simulink model "FullFMS_SIM_V0_1_0_R2025b"  (R2025b)
settings: Solver=FixedStepAuto  StopTime=inf  FixedStep=0.01  MaxStep=0.01  RelTol=1e-2
PreLoadFcn:
  | load("BUS_CONFIG_SIM.mat"); run("Param_SIM_V0_6.m")
values from neighbouring files (symbols this model uses):
  N_PARTS = 3    [Param_SIM_V0_1_2.m]    (also in Param_SIM_V0_1_3.m; Param_SIM_V0_1_4.m; Param_SIM_V0_1_5.m; Param_SIM_V0_1_6.m)
  t_conv = 5    [Param_SIM_V0_1_2.m]    (also in Param_SIM_V0_1_3.m; Param_SIM_V0_1_4.m; Param_SIM_V0_1_5.m; Param_SIM_V0_1_6.m)
  T_CONV_T6 = 3    [Param_SIM_V0_1_2.m]    (also in Param_SIM_V0_1_3.m; Param_SIM_V0_1_4.m; Param_SIM_V0_1_5.m; Param_SIM_V0_1_6.m)
  t_grip = 0.10    (= 0.1)    [Param_SIM_V0_1_2.m]    (also in Param_SIM_V0_1_3.m; Param_SIM_V0_1_4.m; Param_SIM_V0_1_5.m; Param_SIM_V0_1_6.m)
  t_h_cart = 2.38    [Param_SIM_V0_1_2.m]    (also in Param_SIM_V0_1_3.m; Param_SIM_V0_1_4.m; Param_SIM_V0_1_5.m; Param_SIM_V0_1_6.m)
  t_h_del = 2.82    [Param_SIM_V0_1_2.m]    (also in Param_SIM_V0_1_3.m; Param_SIM_V0_1_4.m; Param_SIM_V0_1_5.m; Param_SIM_V0_1_6.m)
  T_HD1_T1 = 2    [Param_SIM_V0_1_2.m]    (also in Param_SIM_V0_1_3.m; Param_SIM_V0_1_4.m; Param_SIM_V0_1_5.m; Param_SIM_V0_1_6.m)
  t_leave = 2    [Param_SIM_V0_1_2.m]    (also in Param_SIM_V0_1_3.m; Param_SIM_V0_1_4.m; Param_SIM_V0_1_5.m; Param_SIM_V0_1_6.m)
  t_sort_clear = 3    [Param_SIM_V0_6.m]
  t_v_down = 0.93    [Param_SIM_V0_1_2.m]    (also in Param_SIM_V0_1_3.m; Param_SIM_V0_1_4.m; Param_SIM_V0_1_5.m; Param_SIM_V0_1_6.m)
  t_v_up = 1.37    [Param_SIM_V0_1_2.m]    (also in Param_SIM_V0_1_3.m; Param_SIM_V0_1_4.m; Param_SIM_V0_1_5.m; Param_SIM_V0_1_6.m)
libraries: opcualib x8
settings Model: SimulationMode=accelerator  PacingRate=0.100000  Creator=guilh  LastModifiedBy=gasie
settings SolverCC: ZeroCrossControl=DisableAll

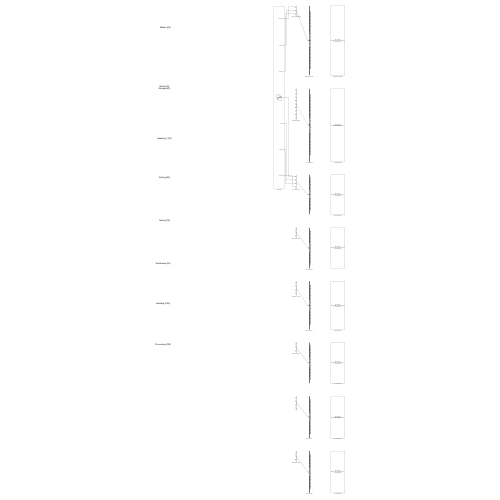
[thumbnail: Simulink's stored preview of the top-level diagram]
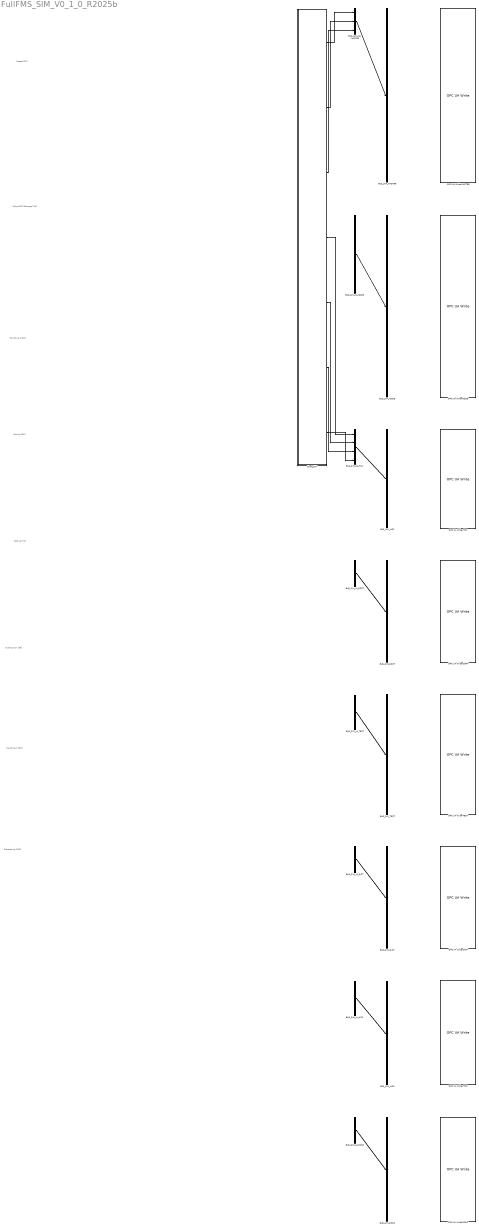
== system FullFMS_SIM_V0_1_0_R2025b ==
  note: Master [20]
  note: Robot [30]
      | Storage [40]
  note: Handling 1 [50]
  note: Sorting [60]
  note: Testing [70]
  note: Distribution [80]
  note: Handling 2 [90]
  note: Processing [100]
  BUS_SIM_DIST : BusSelector  OutputSignals=SimActuators_80.SA_80_Pist_Adv,SimActuators_80.SA_80_Suction_On,SimActuators_80.SA_80_Suction_Off,SimActuators_80.SA_80_Arm_2_Del,SimActuators_80.SA_80_Arm_2_Mag,SimActuators_80.SA_81_Led_Start,SimActuators_80.SA_81_Led_Reset,SimActuators_80.SA_81_Led_Extra1,SimActuators_80.SA_81_Led_Extra2,SimActuators_80.SA_81_Panel_O4,SimActuators_80.SA_81_Panel_O5,SimActuators_80.SA_81_Panel_O6,SimActuators_80.SA_81_Panel_O7,SimControl_80.SC_82_Profibus,SimControl_80.SC_83_RQ_Parts,SimControl_80.SC_85_Initialization,SimControl_80.SC_85_Start,SimControl_80.SC_85_Part_Del,SimControl_80.SC_85_Single,SimControl_80.SC_85_Part_Mag,SimControl_80.SC_85_Continuous,SimControl_80.SC_85_Counted,SimControl_80.SC_86_Mag_Parts,SimControl_80.SC_87_RQ_MParts,SimSensors_80.SS_80_Mag_Full,SimSensors_80.SS_80_Pist_Bck,SimSensors_80.SS_80_Pist_Fwd,SimSensors_80.SS_80_Part_Stuck,SimSensors_80.SS_80_Arm_Mag,SimSensors_80.SS_80_Arm_Del,SimSensors_80.SS_80_Mag_Empty,SimSensors_80.SS_81_Start,SimSensors_80.SS_81_Stop,SimSensors_80.SS_81_Key_Pos,SimSensors_80.SS_81_Reset,SimSensors_80.SS_81_Panel_I4,SimSensors_80.SS_81_Panel_I5,SimSensors_80.SS_81_Panel_I6,SimSensors_80.SS_81_Panel_I7
  BUS_SIM_HD1 : BusSelector  OutputSignals=SimActuators_50.SA_50_Claw_2_Del,SimActuators_50.SA_50_Claw_2_Cart,SimActuators_50.SA_50_Claw_Down,SimActuators_50.SA_50_Close_Claw,SimActuators_50.SA_51_Led_Start,SimActuators_50.SA_51_Led_Reset,SimActuators_50.SA_51_Led_Extra1,SimActuators_50.SA_51_Led_Extra2,SimActuators_50.SA_51_Panel_O4,SimActuators_50.SA_51_Panel_O5,SimActuators_50.SA_51_Panel_O6,SimActuators_50.SA_51_Panel_O7,SimASi_50.SR_53_SortCartID,SimASi_50.SR_54_Request,SimASi_50.SR_54_No_Cart,SimASi_50.SR_54_Cart_Full,SimASi_50.SR_54_CRoute_Out,SimASi_50.SR_54_CRoute_In,SimControl_50.SC_52_Profibus,SimControl_50.SC_55_Initialization,SimControl_50.SC_55_Start,SimControl_50.SC_55_PD_Sort,SimControl_50.SC_55_Cart2Del,SimSensors_50.SS_50_Part_Reserve,SimSensors_50.SS_50_Claw_Cart,SimSensors_50.SS_50_Claw_Del,SimSensors_50.SS_50_Claw_Reserve,SimSensors_50.SS_50_Claw_Low,SimSensors_50.SS_50_Claw_High,SimSensors_50.SS_50_Part_in_Claw,SimSensors_50.SS_51_Start,SimSensors_50.SS_51_Stop,SimSensors_50.SS_51_Key_Pos,SimSensors_50.SS_51_Reset,SimSensors_50.SS_51_Panel_I4,SimSensors_50.SS_51_Panel_I5,SimSensors_50.SS_51_Panel_I6,SimSensors_50.SS_51_Panel_I7
  BUS_SIM_HD2 : BusSelector  OutputSignals=SimActuators_90.SA_90_Claw_2_Cart,SimActuators_90.SA_90_Claw_2_Del,SimActuators_90.SA_90_Claw_Down,SimActuators_90.SA_90_Close_Claw,SimActuators_90.SA_91_Led_Start,SimActuators_90.SA_91_Led_Reset,SimActuators_90.SA_91_Led_Extra1,SimActuators_90.SA_91_Led_Extra2,SimActuators_90.SA_91_Panel_O4,SimActuators_90.SA_91_Panel_O5,SimActuators_90.SA_91_Panel_O6,SimActuators_90.SA_91_Panel_O7,SimASi_90.SR_93_ProcCartID,SimASi_90.SR_94_Request,SimASi_90.SR_94_No_Cart,SimASi_90.SR_94_Cart_Full,SimASi_90.SR_94_CRoute_Out,SimASi_90.SR_94_CRoute_In,SimControl_90.SC_92_Profibus,SimControl_90.SC_95_Initialization,SimControl_90.SC_95_Start,SimControl_90.SC_95_PD_Proc,SimControl_90.SC_95_Cart2Del,SimControl_90.SC_95_PD_Cart,SimControl_90.SC_95_Del2Cart,SimSensors_90.SS_90_Part_Reserve,SimSensors_90.SS_90_Claw_Del,SimSensors_90.SS_90_Claw_Cart,SimSensors_90.SS_90_Claw_Reserve,SimSensors_90.SS_90_Claw_Low,SimSensors_90.SS_90_Claw_High,SimSensors_90.SS_90_Part_in_Claw,SimSensors_90.SS_91_Start,SimSensors_90.SS_91_Stop,SimSensors_90.SS_91_Key_Pos,SimSensors_90.SS_91_Reset,SimSensors_90.SS_91_Panel_I4,SimSensors_90.SS_91_Panel_I5,SimSensors_90.SS_91_Panel_I6,SimSensors_90.SS_91_Panel_I7
  BUS_SIM_IN_DIST : BusCreator  Inputs=3  OutDataTypeStr=Bus: B_SIM_DIST  NonVirtualBus=on
  BUS_SIM_IN_HD1 : BusCreator  Inputs=4  OutDataTypeStr=Bus: B_SIM_HD1  NonVirtualBus=on
  BUS_SIM_IN_HD2 : BusCreator  Inputs=4  OutDataTypeStr=Bus: B_SIM_HD2  NonVirtualBus=on
  BUS_SIM_IN_MASTER : BusCreator  Inputs=3  OutDataTypeStr=Bus: B_SIM_MASTER  NonVirtualBus=on
  BUS_SIM_IN_NODE : BusCreator  Inputs=9  OutDataTypeStr=Bus: B_SIM_NODE  NonVirtualBus=on
  BUS_SIM_IN_PROC : BusCreator  Inputs=3  OutDataTypeStr=Bus: B_SIM_PROC  NonVirtualBus=on
  BUS_SIM_IN_SORT : BusCreator  Inputs=3  OutDataTypeStr=Bus: B_SIM_SORT  NonVirtualBus=on
  BUS_SIM_IN_TEST : BusCreator  Inputs=4  OutDataTypeStr=Bus: B_SIM_TEST  NonVirtualBus=on
  BUS_SIM_MASTER : BusSelector  OutputSignals=SimActuators_20.SA_20_Led_On,SimActuators_20.SA_20_Led_Off,SimActuators_20.SA_20_Conveyor,SimActuators_20.SA_24_Cart_Test,SimActuators_20.SA_25_Cart_Proc,SimActuators_20.SA_26_Cart_Visi,SimActuators_20.SA_27_Cart_Robo,SimActuators_20.SA_28_Cart_Stor,SimActuators_20.SA_29_Cart_Sort,SimControl_20.SC_21_MES_On,SimControl_20.SC_24_Request,SimControl_20.SC_24_CRoute_In,SimControl_20.SC_24_CartDel,SimControl_20.SC_24_CRoute_Out,SimControl_20.SC_25_Request,SimControl_20.SC_25_CRoute_In,SimControl_20.SC_25_CartDel,SimControl_20.SC_25_CRoute_Out,SimControl_20.SC_26_Request,SimControl_20.SC_26_CRoute_In,SimControl_20.SC_26_CartDel,SimControl_20.SC_26_CRoute_Out,SimControl_20.SC_27_Request,SimControl_20.SC_27_CRoute_In,SimControl_20.SC_27_CartDel,SimControl_20.SC_27_CRoute_Out,SimControl_20.SC_28_Request,SimControl_20.SC_28_CRoute_In,SimControl_20.SC_28_CartDel,SimControl_20.SC_28_CRoute_Out,SimControl_20.SC_29_Request,SimControl_20.SC_29_CRoute_In,SimControl_20.SC_29_CartDel,SimControl_20.SC_29_CRoute_Out,SimSensors_20.SS_20_On,SimSensors_20.SS_20_Off,SimSensors_20.SS_20_Controler_On,SimSensors_20.SS_24_Cart_Stat,SimSensors_20.SS_24_Cart_Next,SimSensors_20.SS_24_Optic,SimSensors_20.SS_24_Count,SimSensors_20.SS_24_Pist_Bck,SimSensors_20.SS_25_Cart_Stat,SimSensors_20.SS_25_Cart_Next,SimSensors_20.SS_25_Optic,SimSensors_20.SS_25_Count,SimSensors_20.SS_25_Pist_Bck,SimSensors_20.SS_26_Cart_Stat,SimSensors_20.SS_26_Cart_Next,SimSensors_20.SS_26_Optic,SimSensors_20.SS_26_Count,SimSensors_20.SS_26_Pist_Bck,SimSensors_20.SS_27_Cart_Stat,SimSensors_20.SS_27_Cart_Next,SimSensors_20.SS_27_Optic,SimSensors_20.SS_27_Count,SimSensors_20.SS_27_Pist_Bck,SimSensors_20.SS_28_Cart_Stat,SimSensors_20.SS_28_Cart_Next,SimSensors_20.SS_28_Optic,SimSensors_20.SS_28_Count,SimSensors_20.SS_28_Pist_Bck,SimSensors_20.SS_29_Cart_Stat,SimSensors_20.SS_29_Cart_Next,SimSensors_20.SS_29_Optic,SimSensors_20.SS_29_Count,SimSensors_20.SS_29_Pist_Bck
  BUS_SIM_NODE : BusSelector  OutputSignals=SimActuators_30.SA_30_Led_Start,SimActuators_30.SA_30_Led_Reset,SimActuators_30.SA_30_Led_Extra1,SimActuators_30.SA_30_Led_Extra2,SimActuators_30.SA_30_Spring_Cyl,SimActuators_30.SA_30_Cover_Cyl,SimASi_30.SR_32_RoboCartID,SimASi_30.SR_34_Request,SimASi_30.SR_34_No_Cart,SimASi_30.SR_34_Cart_Full,SimASi_30.SR_34_CRoute_Out,SimASi_30.SR_34_CRoute_In,SimControl_30.SC_30_Robot1,SimControl_30.SC_30_Robot2,SimControl_30.SC_35_Part_Del,SimSensors_30.SS_31_Start,SimSensors_30.SS_31_Stop,SimSensors_30.SS_31_Reset,SimSensors_30.SS_31_Part_in_Claw,SimSensors_30.SS_31_Orientation,SimSensors_30.SS_32_Sp_Cyl_Bck,SimSensors_30.SS_32_Sp_Cyl_Fwd,SimSensors_30.SS_32_Co_Cyl_Bck,SimSensors_30.SS_32_Co_Cyl_Fwd,SimSensors_30.SS_32_Sp_PickUp,SimSensors_30.SS_32_Co_PickUp,SimSensors_30.SS_32_CoMag_Empty,SimRFID_RFID.SID_Ant1_R_TagID,SimRFID_RFID.SID_Ant1_R_UserData,SimRFID_RFID.SID_Ant1_W_TagID,SimRFID_RFID.SID_Ant1_W_UserData,SimRFID_RFID.SID_Ant2_R_TagID,SimRFID_RFID.SID_Ant2_R_UserData,SimRFID_RFID.SID_Ant2_W_TagID,SimRFID_RFID.SID_Ant2_W_UserData,SimRFID_RFID.SID_Ant3_R_TagID,SimRFID_RFID.SID_Ant3_R_UserData,SimRFID_RFID.SID_Ant3_W_TagID,SimRFID_RFID.SID_Ant3_W_UserData,SimRFID_RFID.SID_Ant4_R_TagID,SimRFID_RFID.SID_Ant4_R_UserData,SimRFID_RFID.SID_Ant4_W_TagID,SimRFID_RFID.SID_Ant4_W_UserData,SimActuators_40.SA_41_Led_Start,SimActuators_40.SA_41_Led_Reset,SimActuators_40.SA_41_Led_Extra1,SimActuators_40.SA_41_Led_Extra2,SimActuators_40.SA_41_Panel_O4,SimActuators_40.SA_41_Panel_O5,SimActuators_40.SA_41_Panel_O6,SimActuators_40.SA_41_Panel_O7,SimASi_40.SR_43_StorCartID,SimASi_40.SR_44_Request,SimASi_40.SR_44_No_Cart,SimASi_40.SR_44_Cart_Full,SimASi_40.SR_44_CRoute_Out,SimASi_40.SR_44_CRoute_In,SimControl_40.SC_42_Profibus,SimControl_40.SC_45_Initialization,SimControl_40.SC_45_Start,SimControl_40.SC_45_StorePart,SimControl_40.SC_45_RetrievePart,SimSensors_40.SS_41_Start,SimSensors_40.SS_41_Stop,SimSensors_40.SS_41_Key_Pos,SimSensors_40.SS_41_Reset,SimSensors_40.SS_41_Panel_I4,SimSensors_40.SS_41_Panel_I5,SimSensors_40.SS_41_Panel_I6,SimSensors_40.SS_41_Panel_I7
  BUS_SIM_PROC : BusSelector  OutputSignals=SimActuators_100.SA_100_Drill_On,SimActuators_100.SA_100_RT_On,SimActuators_100.SA_100_Drill_Down,SimActuators_100.SA_100_Drill_Up,SimActuators_100.SA_100_Drill_Pin,SimActuators_100.SA_100_Test_Pin,SimActuators_100.SA_101_Led_Start,SimActuators_100.SA_101_Led_Reset,SimActuators_100.SA_101_Led_Extra1,SimActuators_100.SA_101_Led_Extra2,SimActuators_100.SA_101_Panel_O4,SimActuators_100.SA_101_Panel_O5,SimActuators_100.SA_101_Panel_O6,SimActuators_100.SA_101_Panel_O7,SimControl_100.SC_102_Profibus,SimControl_100.SC_103_RQ_Turns,SimControl_100.SC_105_Initialization,SimControl_100.SC_105_Start,SimControl_100.SC_105_Part_ready,SimControl_100.SC_105_Test,SimControl_100.SC_105_Test_Ok,SimControl_100.SC_105_TestDrill,SimControl_100.SC_105_Test_Fail,SimControl_100.SC_105_Rotation,SimControl_100.SC_106_RT_Counter,SimSensors_100.SS_100_PInit_Pos,SimSensors_100.SS_100_PDrill_Pos,SimSensors_100.SS_100_PTest_Pos,SimSensors_100.SS_100_SDrill_High,SimSensors_100.SS_100_SDrill_Low,SimSensors_100.SS_100_RT_Sensor,SimSensors_100.SS_100_PTest_Ok,SimSensors_100.SS_101_Start,SimSensors_100.SS_101_Stop,SimSensors_100.SS_101_Key_Pos,SimSensors_100.SS_101_Reset,SimSensors_100.SS_101_Panel_I4,SimSensors_100.SS_101_Panel_I5,SimSensors_100.SS_101_Panel_I6,SimSensors_100.SS_101_Panel_I7
  BUS_SIM_SORT : BusSelector  OutputSignals=SimActuators_60.SA_60_Conveyor,SimActuators_60.SA_60_P1,SimActuators_60.SA_60_P2,SimActuators_60.SA_60_Identify,SimActuators_60.SA_61_Led_Start,SimActuators_60.SA_61_Led_Reset,SimActuators_60.SA_61_Led_Extra1,SimActuators_60.SA_61_Led_Extra2,SimActuators_60.SA_61_Panel_O4,SimActuators_60.SA_61_Panel_O5,SimActuators_60.SA_61_Panel_O6,SimActuators_60.SA_61_Panel_O7,SimControl_60.SC_62_Profibus,SimControl_60.SC_65_Initialization,SimControl_60.SC_65_RBS_Output,SimControl_60.SC_65_ID_1,SimControl_60.SC_65_RSB_Output,SimControl_60.SC_65_ID_2,SimControl_60.SC_65_BRS_Output,SimControl_60.SC_65_Part_Sorted,SimControl_60.SC_65_BSR_Output,SimControl_60.SC_65_SRB_Output,SimControl_60.SC_65_SBR_Output,SimSensors_60.SS_60_SPart,SimSensors_60.SS_60_SInd,SimSensors_60.SS_60_SPhoto,SimSensors_60.SS_60_Part_Pass,SimSensors_60.SS_60_SL1_Bck,SimSensors_60.SS_60_SL1_Fwd,SimSensors_60.SS_60_SL2_Bck,SimSensors_60.SS_60_SL2_Fwd,SimSensors_60.SS_61_Start,SimSensors_60.SS_61_Stop,SimSensors_60.SS_61_Key_Pos,SimSensors_60.SS_61_Reset,SimSensors_60.SS_61_Panel_I4,SimSensors_60.SS_61_Panel_I5,SimSensors_60.SS_61_Panel_I6,SimSensors_60.SS_61_Panel_I7
  BUS_SIM_TEST : BusSelector  OutputSignals=SimActuators_70.SA_70_Elev_Down,SimActuators_70.SA_70_Elev_Up,SimActuators_70.SA_70_Eject_Part,SimActuators_70.SA_70_Air_On,SimActuators_70.SA_71_Led_Start,SimActuators_70.SA_71_Led_Reset,SimActuators_70.SA_71_Led_Extra1,SimActuators_70.SA_71_Led_Extra2,SimActuators_70.SA_71_Panel_O4,SimActuators_70.SA_71_Panel_O5,SimActuators_70.SA_71_Panel_O6,SimActuators_70.SA_71_Panel_O7,SimASi_70.SR_73_TestCartID,SimASi_70.SR_74_Request,SimASi_70.SR_74_No_Cart,SimASi_70.SR_74_Cart_Full,SimASi_70.SR_74_CRoute_Out,SimASi_70.SR_74_CRoute_In,SimControl_70.SC_72_Profibus,SimControl_70.SC_75_Initialization,SimControl_70.SC_75_RQ_Delivery1,SimControl_70.SC_75_ID_Delivery1,SimControl_70.SC_75_RQ_Delivery2,SimControl_70.SC_75_ID_Delivery2,SimControl_70.SC_75_Identified,SimControl_70.SC_75_Part_Del,SimControl_70.SC_75_Requested,SimControl_70.SC_75_RQ_Part_Del,SimControl_70.SC_75_RQ_Wrong,SimControl_70.SC_75_Identified80,SimControl_70.SC_75_Requested80,SimSensors_70.SS_70_SInductive,SimSensors_70.SS_70_SPart,SimSensors_70.SS_70_SStation,SimSensors_70.SS_70_SPart_Height,SimSensors_70.SS_70_Elev_High,SimSensors_70.SS_70_Elev_Low,SimSensors_70.SS_70_Pist_Bck,SimSensors_70.SS_71_Start,SimSensors_70.SS_71_Stop,SimSensors_70.SS_71_Key_Pos,SimSensors_70.SS_71_Reset,SimSensors_70.SS_71_Panel_I4,SimSensors_70.SS_71_Panel_I5,SimSensors_70.SS_71_Panel_I6,SimSensors_70.SS_71_Panel_I7
  Chart_SIM : Stateflow chart  TreatAsAtomicUnit=on
  OPC UA Write-DIST : opcualib/OPC UA Write  SelectedServer=AAS OPC Distribution  ServerList=AAS OPC Distribution  NodeList={}  SampleTime=-1
  OPC UA Write-HD1 : opcualib/OPC UA Write  SelectedServer=AAS OPC Handling1  ServerList=AAS OPC Handling1  NodeList={}  SampleTime=-1
  OPC UA Write-HD2 : opcualib/OPC UA Write  SelectedServer=AAS OPC Handling2  ServerList=AAS OPC Handling2  NodeList={}  SampleTime=-1
  OPC UA Write-MASTER : opcualib/OPC UA Write  SelectedServer=AAS OPC Master  ServerList=AAS OPC Master  NodeList={}  SampleTime=-1
  OPC UA Write-NODE : opcualib/OPC UA Write  SelectedServer=AAS Server Robot+Storage  ServerList=AAS Server Robot+Storage  NodeList={}  SampleTime=-1
  OPC UA Write-PROC : opcualib/OPC UA Write  SelectedServer=AAS OPC Processing  ServerList=AAS OPC Processing  NodeList={}  SampleTime=-1
  OPC UA Write-SORT : opcualib/OPC UA Write  SelectedServer=AAS OPC Sorting  ServerList=AAS OPC Sorting  NodeList={}  SampleTime=-1
  OPC UA Write-TEST : opcualib/OPC UA Write  SelectedServer=AAS OPC Testing  ServerList=AAS OPC Testing  NodeList={}  SampleTime=-1
  wires:
  BUS_SIM_IN_MASTER/1 -> BUS_SIM_MASTER/1
  BUS_SIM_IN_NODE/1 -> BUS_SIM_NODE/1
  BUS_SIM_IN_HD1/1 -> BUS_SIM_HD1/1
  BUS_SIM_IN_SORT/1 -> BUS_SIM_SORT/1
  BUS_SIM_IN_TEST/1 -> BUS_SIM_TEST/1
  BUS_SIM_IN_DIST/1 -> BUS_SIM_DIST/1
  BUS_SIM_IN_HD2/1 -> BUS_SIM_HD2/1
  BUS_SIM_IN_PROC/1 -> BUS_SIM_PROC/1
  Chart_SIM/1(SimActuators_20) -> BUS_SIM_IN_MASTER/1
  Chart_SIM/2(SimControl_20) -> BUS_SIM_IN_MASTER/2
  Chart_SIM/3(SimSensors_20) -> BUS_SIM_IN_MASTER/3
  Chart_SIM/4(SimActuators_50) -> BUS_SIM_IN_HD1/1
  Chart_SIM/5(SimASi_50) -> BUS_SIM_IN_HD1/2
  Chart_SIM/6(SimControl_50) -> BUS_SIM_IN_HD1/3
  Chart_SIM/7(SimSensors_50) -> BUS_SIM_IN_HD1/4

== stateflow chart FullFMS_SIM_V0_1_0_R2025b/Chart_SIM ==
  settings: updateMethod=DISCRETE  sampleTime=Ts_SIM
  state Conveyor29 [parallel]
    settings: executionOrder=1
    state Idle
      entry: SimSensors_20.SS_29_Cart_Stat=false; SimSensors_20.SS_29_Optic=false; SimSensors_20.SS_29_Cart_Next=false;
    state Arriving
      entry: SimSensors_20.SS_29_Cart_Next=true; SimActuators_20.SA_20_Conveyor=true; SimSensors_20.SS_20_Controler_On=true;
    state AtStop
      entry: SimSensors_20.SS_29_Cart_Next=false; SimSensors_20.SS_29_Count=true; SimSensors_20.SS_29_Cart_Stat=true; SimSensors_20.SS_29_Optic=true;
      PartOnCart=true; CartAt29=true; SimActuators_20.SA_20_Conveyor=false;
    state Delivered
      entry: SimSensors_20.SS_29_Count=false; SimControl_20.SC_29_CartDel=true; CRouteIn54=true; SimASi_50.SR_54_CRoute_In=true;
      during: SimSensors_20.SS_29_Optic = PartOnCart;
    state Leaving
      entry: SimControl_20.SC_29_CartDel=false; CRouteIn54=false; SimASi_50.SR_54_CRoute_In=false; CartAt29=false;
    (default) -> Idle
    Leaving -> Idle : after(t_leave,sec)
    Idle -> Arriving : [nDone < N_PARTS]
    Arriving -> AtStop : after(t_conv,sec)
    AtStop -> Delivered : after(T_CONV_T6,sec)
    Delivered -> Leaving : [SimASi_50.SR_54_CRoute_Out]
  state HD1_Ctrl [parallel]
    settings: executionOrder=2
    state Init
      entry: SimControl_50.SC_52_Profibus=true; SimControl_50.SC_55_PD_Sort=false; SimASi_50.SR_54_CRoute_Out=false;
      SimActuators_50.SA_50_Claw_Down=false; SimActuators_50.SA_50_Close_Claw=false; SimActuators_50.SA_50_Claw_2_Del=false; SimActuators_50.SA_50_Claw_2_Cart=false;
    state Ready
      entry: SimControl_50.SC_55_Initialization=true;
    state N1_StartMove
      entry: SimControl_50.SC_55_PD_Sort=false;
    state N2_LowerClaw
      entry: SimActuators_50.SA_50_Claw_Down=true;
    state N3_CloseClaw
      entry: SimActuators_50.SA_50_Close_Claw=true;
    state N3_Raise
      entry: SimActuators_50.SA_50_Claw_Down=false;
    state N4_Claw2Del
      entry: SimActuators_50.SA_50_Claw_2_Cart=false; SimActuators_50.SA_50_Claw_2_Del=true;
    state N5_LowerClaw2
      entry: SimActuators_50.SA_50_Claw_Down=true;
    state N6_Release
      entry: SimActuators_50.SA_50_Close_Claw=false;
    state N6_Raise
      entry: SimActuators_50.SA_50_Claw_Down=false;
    state N7_PDSort
      entry: SimControl_50.SC_55_PD_Sort=true;
    state N8_Claw2Cart
      entry: SimActuators_50.SA_50_Claw_2_Del=false; SimActuators_50.SA_50_Claw_2_Cart=true; Claw2CartCmd=true;
    state N9_CRouteOut
      entry: SimActuators_50.SA_50_Claw_2_Cart=false; Claw2CartCmd=false; SimASi_50.SR_54_CRoute_Out=true;
      exit: SimASi_50.SR_54_CRoute_Out=false; nDone = nDone + 1;
    (default) -> Init
    Init -> Ready : [SimSensors_50.SS_50_Claw_Cart && SimSensors_50.SS_50_Claw_High && ~SimSensors_50.SS_50_Part_in_Claw]
    N9_CRouteOut -> Ready : after(T_HD1_T1,sec)
    Ready -> N1_StartMove : [CRouteIn54 && CartAt29 && SimSensors_20.SS_29_Optic && ~SPart60]
    N1_StartMove -> N2_LowerClaw : [~SimControl_50.SC_55_PD_Sort && SimSensors_50.SS_50_Claw_Cart && SimSensors_50.SS_50_Claw_High && ~SimSensors_50.SS_50_Part_in_Claw]
    N2_LowerClaw -> N3_CloseClaw : [SimSensors_50.SS_50_Claw_Cart && SimSensors_50.SS_50_Claw_Low]
    N3_CloseClaw -> N3_Raise : [SimSensors_50.SS_50_Part_in_Claw]
    N3_Raise -> N4_Claw2Del : [SimSensors_50.SS_50_Claw_High && SimSensors_50.SS_50_Part_in_Claw && ~SimSensors_50.SS_50_Claw_Del]
    N4_Claw2Del -> N5_LowerClaw2 : [SimSensors_50.SS_50_Claw_Del && SimSensors_50.SS_50_Claw_High && SimSensors_50.SS_50_Part_in_Claw]
    N5_LowerClaw2 -> N6_Release : [SimSensors_50.SS_50_Claw_Del && SimSensors_50.SS_50_Claw_Low]
    N6_Release -> N6_Raise : [~SimSensors_50.SS_50_Part_in_Claw]
    N6_Raise -> N7_PDSort : [SimSensors_50.SS_50_Claw_Del && SimSensors_50.SS_50_Claw_High && ~SimSensors_50.SS_50_Part_in_Claw]
    N7_PDSort -> N8_Claw2Cart
    N8_Claw2Cart -> N9_CRouteOut : [SimSensors_50.SS_50_Claw_Cart]
  state HD1_Plant [parallel]
    settings: executionOrder=3
    state Vertical [parallel]
      settings: executionOrder=1
      state High
        entry: SimSensors_50.SS_50_Claw_High=true; SimSensors_50.SS_50_Claw_Low=false;
      state GoingDown
        entry: SimSensors_50.SS_50_Claw_High=false;
      state Low
        entry: SimSensors_50.SS_50_Claw_Low=true;
      state GoingUp
        entry: SimSensors_50.SS_50_Claw_Low=false;
      (default) -> High
      GoingUp -> High [order 1] : after(t_v_up,sec)
      High -> GoingDown : [SimActuators_50.SA_50_Claw_Down]
      GoingUp -> GoingDown [order 2] : [SimActuators_50.SA_50_Claw_Down]
      GoingDown -> Low [order 1] : after(t_v_down,sec)
      GoingDown -> GoingUp [order 2] : [~SimActuators_50.SA_50_Claw_Down]
      Low -> GoingUp : [~SimActuators_50.SA_50_Claw_Down]
    state Horizontal [parallel]
      settings: executionOrder=2
      state AtCart
        entry: SimSensors_50.SS_50_Claw_Cart=true; SimSensors_50.SS_50_Claw_Del=false;
      state ToDel
        entry: SimSensors_50.SS_50_Claw_Cart=false;
      state AtDel
        entry: SimSensors_50.SS_50_Claw_Del=true;
      state ToCart
        entry: SimSensors_50.SS_50_Claw_Del=false;
      (default) -> AtCart
      ToCart -> AtCart : after(t_h_cart,sec)
      AtCart -> ToDel : [SimActuators_50.SA_50_Claw_2_Del]
      ToDel -> AtDel : after(t_h_del,sec)
      AtDel -> ToCart : [SimActuators_50.SA_50_Claw_2_Cart]
    state Gripper [parallel]
      settings: executionOrder=3
      state Empty
        entry: SimSensors_50.SS_50_Part_in_Claw=false;
      state Gripping
      state Holding
        entry: SimSensors_50.SS_50_Part_in_Claw=true; PartOnCart=false;
      state Releasing
      (default) -> Empty
      Releasing -> Empty : after(t_grip,sec){SPart60 = SimSensors_50.SS_50_Claw_Del;}
      Empty -> Gripping : [SimActuators_50.SA_50_Close_Claw && SimSensors_50.SS_50_Claw_Low && SimSensors_50.SS_50_Claw_Cart && PartOnCart]
      Gripping -> Holding : after(t_grip,sec)
      Holding -> Releasing : [~SimActuators_50.SA_50_Close_Claw && SimSensors_50.SS_50_Claw_Low]
    state SortingFeed [parallel]
      settings: executionOrder=4
      state NoPart
      state HasPart
      (default) -> NoPart
      HasPart -> NoPart : after(t_sort_clear,sec){SPart60 = false;}
      NoPart -> HasPart : [SPart60]
  data: SimActuators_20 output Bus: B_SimActuators_20; SimControl_20 output Bus: B_SimControl_20; SimSensors_20 output Bus: B_SimSensors_20; SimActuators_50 output Bus: B_SimActuators_50; SimASi_50 output Bus: B_SimASi_50; SimControl_50 output Bus: B_SimControl_50; SimSensors_50 output Bus: B_SimSensors_50; T_HD1_T1 parameter double; T_CONV_T6 parameter double; t_v_down parameter double; t_v_up parameter double; t_h_del parameter double; t_h_cart parameter double; t_grip parameter double; t_conv parameter double; t_leave parameter double; t_sort_clear parameter double; N_PARTS parameter double; SPart60 local boolean =false; PartOnCart local boolean =false; CartAt29 local boolean =false; CRouteIn54 local boolean =false; Claw2CartCmd local boolean =false; nDone local double =0
